simulink model "ECG_Rhythm_PVC_Detection_v2_"  (R2019a)
settings: Solver=FixedStepDiscrete  StartTime=0.0  StopTime=30  FixedStep=1/360  RelTol=1e-3
libraries: simulink x5, dspfdesign x2, dspstat3 x1
settings Model: Creator=atif  LastModifiedBy=Admin

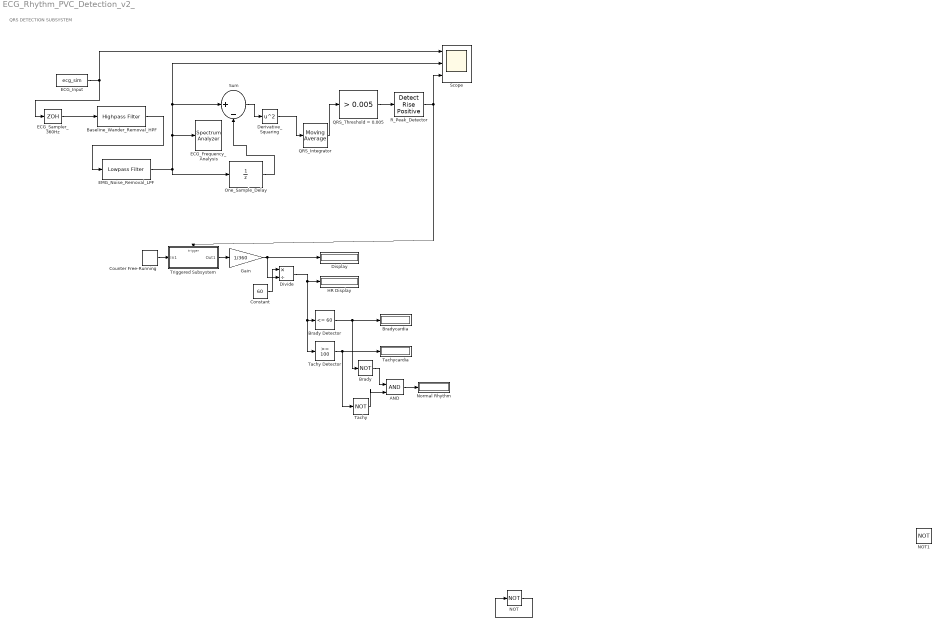
== system ECG_Rhythm_PVC_Detection_v2_ ==
  note: QRS DETECTION SUBSYSTEM
  AND : Logic  IconShape=distinctive  AllPortsSameDT=off  OutDataTypeStr=boolean
  Baseline_Wander_Removal_HPF : dspfdesign/Highpass Filter  FilterType=FIR  DesignForMinimumOrder=on  FilterOrder=50  StopbandFrequency=0.1  PassbandFrequency=0.5  StopbandAttenuation=80  PassbandRipple=0.1  InheritSampleRate=off  SampleRate=360  SimulateUsing=Interpreted execution  roundingMode=Floor  coeffsDataTypeStr=fixdt(1,16)
      settings: SourceProductName=DSP System Toolbox
  Brady : Logic  Operator=NOT  IconShape=distinctive  AllPortsSameDT=off  OutDataTypeStr=boolean
  Brady Detector : simulink/Logic and Bit Operations/Compare To Constant  relop=<=  const=60  OutDataTypeStr=boolean
  Bradycardia : Display
  Constant : Constant  Value=60
  Counter Free-Running : simulink/Sources/Counter Free-Running  NumBits=32  tsamp=1/360
  Derivative_Squaring : Math  Operator=square  SaturateOnIntegerOverflow=on
  Display : Display
  Divide : Product  Inputs=*/
  ECG_Frequency_Analysis : SpectrumAnalyzer
  ECG_Input : FromWorkspace  VariableName=ecg_sim  SampleTime=0  Interpolate=off  OutputAfterFinalValue=Holding final value
  ECG_Sampler_360Hz : ZeroOrderHold  SampleTime=1/360
  EMG_Noise_Removal_LPF : dspfdesign/Lowpass Filter  FilterType=FIR  DesignForMinimumOrder=on  FilterOrder=50  PassbandFrequency=40  StopbandFrequency=45  PassbandRipple=0.1  StopbandAttenuation=80  InheritSampleRate=off  SampleRate=360  SimulateUsing=Interpreted execution  roundingMode=Floor  coeffsDataTypeStr=fixdt(1,16)
  Gain : Gain  Gain=1/360
  HR Display : Display
  NOT : Logic  Operator=NOT  IconShape=distinctive  AllPortsSameDT=off  OutDataTypeStr=boolean
  NOT1 : Logic  Operator=NOT  IconShape=distinctive  AllPortsSameDT=off  OutDataTypeStr=boolean
  Normal Rhythm : Display
  One_Sample_Delay : UnitDelay  SampleTime=1/360  HasFrameUpgradeWarning=on
  QRS_Integrator : dspstat3/Moving Average  Method=Sliding window  ForgettingFactorPort=off  SpecifyWindowLength=on  WindowLength=54  ForgettingFactor=0.9  SimulateUsing=Code generation
  QRS_Threshold = 0.005 : simulink/Logic and Bit Operations/Compare To Constant  relop=>  const=0.005  OutDataTypeStr=boolean
  R_Peak_Detector : simulink/Logic and Bit Operations/Detect Rise Positive  vinit=0  OutDataTypeStr=boolean
  Scope : Scope  NumInputPorts=3
  Sum : Sum  Inputs=|+-
  Tachy : Logic  Operator=NOT  IconShape=distinctive  AllPortsSameDT=off  OutDataTypeStr=boolean
  Tachy Detector : simulink/Logic and Bit Operations/Compare To Constant  relop=>=  const=100  OutDataTypeStr=boolean
  Tachycardia : Display
  Triggered Subsystem : Subsystem  TreatAsAtomicUnit=on
  wires:
  ECG_Input/1 -> ECG_Sampler_360Hz/1, Scope/1
  Baseline_Wander_Removal_HPF/1 -> EMG_Noise_Removal_LPF/1
  ECG_Sampler_360Hz/1 -> Baseline_Wander_Removal_HPF/1
  One_Sample_Delay/1 -> Sum/2
  EMG_Noise_Removal_LPF/1 -> Scope/2, Sum/1, ECG_Frequency_Analysis/1, One_Sample_Delay/1
  Sum/1 -> Derivative_Squaring/1
  QRS_Integrator/1 -> QRS_Threshold = 0.005/1
  Derivative_Squaring/1 -> QRS_Integrator/1
  QRS_Threshold = 0.005/1 -> R_Peak_Detector/1
  R_Peak_Detector/1 -> Triggered Subsystem/Trigger, Scope/3
  Counter Free-Running/1 -> Triggered Subsystem/1(In1)
  Triggered Subsystem/1(Out1) -> Gain/1
  Gain/1 -> Display/1, Divide/2
  Constant/1 -> Divide/1
  Divide/1 -> Brady Detector/1, Tachy Detector/1, HR Display/1
  Brady Detector/1 -> Bradycardia/1, Brady/1
  Tachy Detector/1 -> Tachycardia/1, Tachy/1
  NOT/1 -> NOT/1
  Tachy/1 -> AND/2
  Brady/1 -> AND/1
  AND/1 -> Normal Rhythm/1

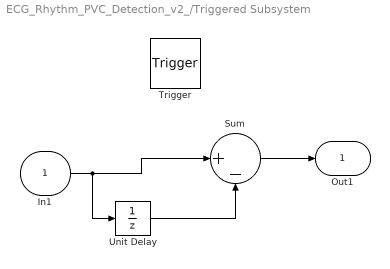
== system ECG_Rhythm_PVC_Detection_v2_/Triggered Subsystem ==
  In1 : Inport
  Trigger : TriggerPort  VariantControl=Variant
  Sum : Sum  Inputs=|+-
  Unit Delay : UnitDelay  SampleTime=-1  HasFrameUpgradeWarning=on
  Out1 : Outport
  wires:
  In1/1 -> Unit Delay/1, Sum/1
  Unit Delay/1 -> Sum/2
  Sum/1 -> Out1/1
